simulink model "SourceBinaire"  (R2023b)
settings: Solver=FixedStepDiscrete  StartTime=0.0  StopTime=1e5-1  FixedStep=Tb  RelTol=1e-3
undefined symbols (not defined in the file or in its folder): graine, p1, Tb
settings Model: Creator=e2405714  LastModifiedBy=e2405714

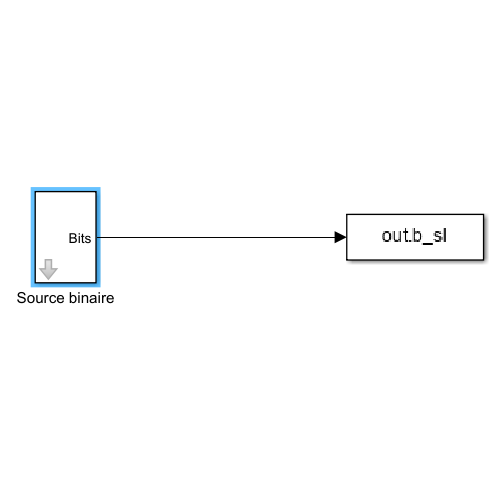
[thumbnail: Simulink's stored preview of the top-level diagram]
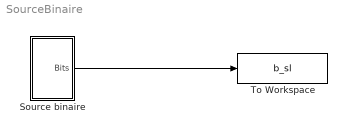
== system SourceBinaire ==
  Source binaire : Subsystem  mask{p1=p1, Tb=Tb, graine=graine}
      mask prompts: p1 "Probabilité d'émettre un 1"; Tb "Durée bit"
  To Workspace : ToWorkspace  VariableName=b_sl  SampleTime=-1
  wires:
  Source binaire/1(Bits) -> To Workspace/1

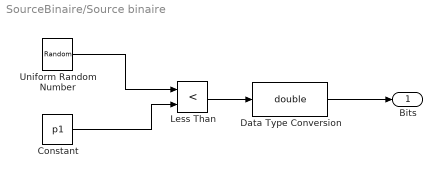
== system SourceBinaire/Source binaire ==
  Constant : Constant  Value=p1  SampleTime=Tb
  Data Type Conversion : DataTypeConversion  OutDataTypeStr=double  SaturateOnIntegerOverflow=off  RndMeth=Floor
  Less Than : RelationalOperator  Operator=<  OutDataTypeStr=boolean  RndMeth=Simplest  InputSameDT=off
  Uniform Random Number : UniformRandomNumber  Minimum=0  Seed=graine  SampleTime=Tb
  Bits : Outport
  wires:
  Less Than/1 -> Data Type Conversion/1
  Constant/1 -> Less Than/2
  Data Type Conversion/1 -> Bits/1
  Uniform Random Number/1 -> Less Than/1
